simulink model "rl_top"  (Simulink 10.3)
settings: Solver=ode23t  StartTime=0.0  StopTime=2  RelTol=0.001
libraries: simulink x14, rllib x1
settings Model: Creator=root  LastModifiedBy=User  MultithreadedSim=on
settings SolverCC: ConsecutiveZCsStepRelTol=2.8421709430404e-13
settings DataIOCC: SignalLoggingSaveFormat=Dataset  SaveOutput=off  SignalLogging=off  DSMLogging=off  SaveTime=off
settings OptimizationCC: ExpressionDepthLimit=128  LifeSpan=auto
settings DebuggingCC: UnderspecifiedInitializationDetection=Simplified  MergeDetectMultiDrivingBlocksExec=error  FcnCallInpInsideContextMsg=error  StateNameClashWarn=none  SFUnexpectedBacktrackingDiag=error  SFNoUnconditionalDefaultTransitionDiag=error  SFExecutionAtInitializationDiag=warning
settings HardwareCC: ProdBitPerPointer=64  ProdBitPerSizeT=64  ProdBitPerPtrDiffT=64  ProdLargestAtomicFloat=Float  ProdIntDivRoundTo=Zero  ProdEndianess=LittleEndian  ProdWordSize=64  ProdHWDeviceType=Intel->x86-64 (Windows64)
settings ModelReferenceCC: PropagateSignalLabelsOutOfModel=on
settings SFSimCC: SimUseLocalCustomCode=on
settings RTWCC: RTWUseLocalCustomCode=on
settings CodeAppCC: StateflowObjectComments=off
settings GRTTargetCC: TargetLangStandard=C99 (ISO)  CombineOutputUpdateFcns=on  GRTInterface=off
settings ConfigComp: CovMetricSettings=dwe  CovSaveCumulativeToWorkspaceVar=off  CovSaveSingleToWorkspaceVar=off  CovExternalEMLEnable=on

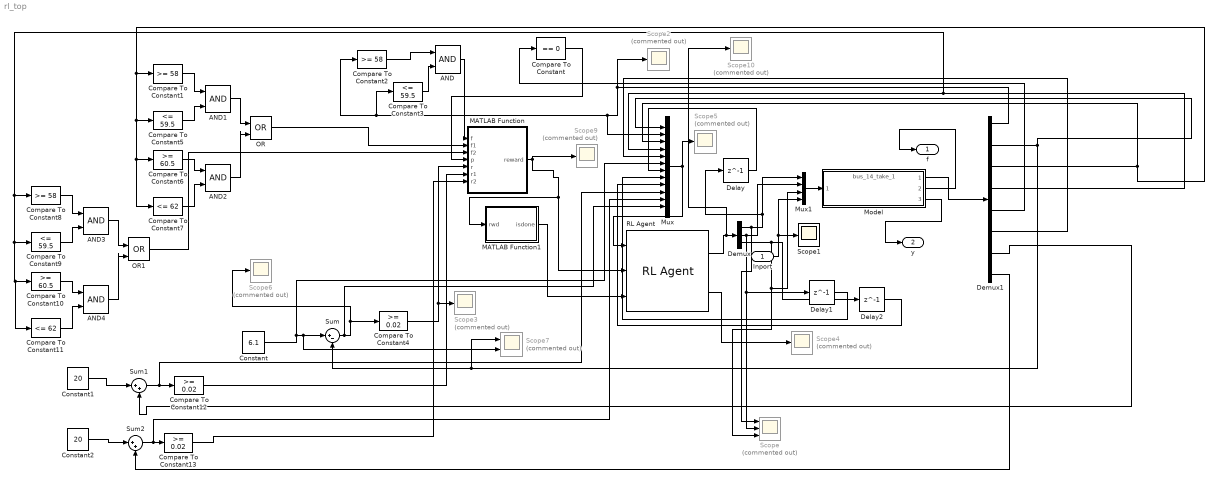
== system rl_top ==
  Inport : Inport
  AND{,1..4} (5 alike) : Logic  IconShape=distinctive  AllPortsSameDT=off  OutDataTypeStr=boolean
  Compare To Constant : simulink/Logic and Bit Operations/Compare To Constant  relop===  const=0  OutDataTypeStr=boolean
  Compare To Constant1 : simulink/Logic and Bit Operations/Compare To Constant  relop=>=  const=58  OutDataTypeStr=boolean
  Compare To Constant10 : simulink/Logic and Bit Operations/Compare To Constant  relop=>=  const=60.5  OutDataTypeStr=boolean
  Compare To Constant11 : simulink/Logic and Bit Operations/Compare To Constant  relop=<=  const=62  OutDataTypeStr=boolean
  Compare To Constant12 : simulink/Logic and Bit Operations/Compare To Constant  relop=>=  const=0.02  OutDataTypeStr=boolean
  Compare To Constant13 : simulink/Logic and Bit Operations/Compare To Constant  relop=>=  const=0.02  OutDataTypeStr=boolean
  Compare To Constant2 : simulink/Logic and Bit Operations/Compare To Constant  relop=>=  const=58  OutDataTypeStr=boolean
  Compare To Constant3 : simulink/Logic and Bit Operations/Compare To Constant  relop=<=  const=59.5  OutDataTypeStr=boolean
  Compare To Constant4 : simulink/Logic and Bit Operations/Compare To Constant  relop=>=  const=0.02  OutDataTypeStr=boolean
  Compare To Constant5 : simulink/Logic and Bit Operations/Compare To Constant  relop=<=  const=59.5  OutDataTypeStr=boolean
  Compare To Constant6 : simulink/Logic and Bit Operations/Compare To Constant  relop=>=  const=60.5  OutDataTypeStr=boolean
  Compare To Constant7 : simulink/Logic and Bit Operations/Compare To Constant  relop=<=  const=62  OutDataTypeStr=boolean
  Compare To Constant8 : simulink/Logic and Bit Operations/Compare To Constant  relop=>=  const=58  OutDataTypeStr=boolean
  Compare To Constant9 : simulink/Logic and Bit Operations/Compare To Constant  relop=<=  const=59.5  OutDataTypeStr=boolean
  Constant : Constant  Value=6.1
  Constant1 : Constant  Value=20
  Constant2 : Constant  Value=20
  Delay : Delay  DelayLength=1
  Delay1 : Delay  DelayLength=1
  Delay2 : Delay  DelayLength=1
  Demux : Demux  Outputs=3
  Demux1 : Demux  Outputs=8
  MATLAB Function : MATLAB Function  TreatAsAtomicUnit=on
  MATLAB Function1 : MATLAB Function  TreatAsAtomicUnit=on
  Model : ModelReference  ModelNameDialog=bus_14_take_1  SimulationMode=Normal  ModelReferenceVersion=1.46
  Mux : Mux  Inputs=12
  Mux1 : Mux
  OR : Logic  Operator=OR  IconShape=distinctive  AllPortsSameDT=off  OutDataTypeStr=boolean
  OR1 : Logic  Operator=OR  IconShape=distinctive  AllPortsSameDT=off  OutDataTypeStr=boolean
  RL Agent : rllib/RL Agent  Agent=agent1  ExternalActionAsInput=off  ProvideCumRwd=on  TreatAsDirectFeedthrough=on
  Scope : Scope  Commented=on  NumInputPorts=3
  Scope1 : Scope
  Scope{2..6,9..10} (7 alike) : Scope  Commented=on
  Scope7 : Scope  Commented=on  NumInputPorts=2
  Sum : Sum  Inputs=|+-
  Sum1 : Sum  Inputs=|++
  Sum2 : Sum  Inputs=|++
  f : Outport
  y : Outport  Port=2
  wires:
  Demux1/1 -> Compare To Constant3/1, Compare To Constant2/1, Mux/2, Scope2/1
  Demux1/5 -> Compare To Constant/1
  Compare To Constant/1 -> MATLAB Function/4(p)
  AND/1 -> MATLAB Function/1(f)
  MATLAB Function/1(reward) -> Scope9/1, RL Agent/2, MATLAB Function1/1(rwd)
  MATLAB Function1/1(isdone) -> RL Agent/3
  Mux/1 -> RL Agent/1, Scope5/1
  RL Agent/2 -> Scope4/1
  Demux1/3 -> Compare To Constant7/1, Compare To Constant6/1, Compare To Constant5/1, Compare To Constant1/1, Mux/3
  Demux1/4 -> Compare To Constant11/1, Compare To Constant10/1, Compare To Constant9/1, Compare To Constant8/1, Mux/4
  Demux1/6 -> Mux/5
  Compare To Constant3/1 -> AND/2
  Compare To Constant2/1 -> AND/1
  Demux1/2 -> Mux/1, Scope7/1, Sum/2
  Sum/1 -> Mux/12, Scope6/1, Compare To Constant4/1
  Compare To Constant4/1 -> Scope3/1, MATLAB Function/5(r)
  Constant/1 -> Mux/6, Scope7/2, Sum/1
  Delay/1 -> Mux/7
  Demux/3 -> Mux1/3, Scope/3, Delay2/1
  RL Agent/1 -> Scope10/1, Demux/1
  Demux/1 -> Scope/1, Mux1/1, Delay/1
  Demux/2 -> Mux1/2, Delay1/1, Scope/2
  Delay1/1 -> Mux/8
  Delay2/1 -> Mux/9
  Compare To Constant5/1 -> AND1/2
  Compare To Constant1/1 -> AND1/1
  Compare To Constant6/1 -> AND2/1
  Compare To Constant7/1 -> AND2/2
  AND1/1 -> OR/1
  AND2/1 -> OR/2
  Compare To Constant8/1 -> AND3/1
  Compare To Constant9/1 -> AND3/2
  AND4/1 -> OR1/2
  Compare To Constant11/1 -> AND4/2
  AND3/1 -> OR1/1
  Compare To Constant10/1 -> AND4/1
  OR/1 -> MATLAB Function/2(f1)
  OR1/1 -> MATLAB Function/3(f2)
  Demux1/8 -> Sum2/2
  Constant1/1 -> Sum1/1
  Constant2/1 -> Sum2/1
  Sum1/1 -> Mux/10, Compare To Constant12/1
  Sum2/1 -> Mux/11, Compare To Constant13/1
  Compare To Constant12/1 -> MATLAB Function/6(r1)
  Compare To Constant13/1 -> MATLAB Function/7(r2)
  Inport/1 -> Scope1/1, Mux1/4
  Demux1/7 -> Sum1/2
  Mux1/1 -> Model/1
  Model/1 -> Demux1/1
  Model/2 -> f/1
  Model/3 -> y/1

== matlab function MATLAB Function ==
  data: f input double; f1 input double; f2 input double; p input double; reward output double; r input double; r1 input double; r2 input double
function reward = fcn(f,f1,f2,p,r,r1,r2)
if (f==1&&f1==1&&f2==1&&r==1&&r1==1&&r2==1)
    reward=6;
elseif(f ==1 && r==1)
  reward=4;
elseif(f1==1&&r1==1)
    reward=3;
    elseif(f2==1&&r2==1)
     reward=3;
     elseif(p==1&&(f==1||f1==1||f2==1))
          reward=1.5;
           elseif(p==1&&(r==1||r1==1||r2==1))
          reward=2;
    else
        
     reward=-6;   
end

== matlab function MATLAB Function1 ==
  data: rwd input double; isdone output double
function isdone = fcn(rwd)

if (abs(rwd) >50)
    isdone=1;
else
  isdone=0;
end
